simulink model "W09_E4_Bandwidth"  (R2024b)
settings: Solver=ode45  StartTime=0.0  StopTime=t_end  MaxStep=0.02  RelTol=1e-3
PreLoadFcn:
  | % W09_E4_Bandwidth 기본 파라미터 (모델을 열 때 자동 실행)
  | defs = { 'K',0.5 ; 'w_in',0.4 ; 't_end',120 ;
  |          'numG',1 ; 'denG',[1 2 1 0] };
  | for ii = 1:size(defs,1)
  |     if ~evalin('base', sprintf('exist(''%s'',''var'')', defs{ii,1}))
  |         assignin('base', defs{ii,1}, defs{ii,2});
  |     end
  | end
  | clear defs ii
values from neighbouring files (symbols this model uses):
  K = 0.5    [W09_02_pm_to_time.m]    (also in W09_03_run_simulink.m; W09_07_examples.m)
  w_in = w_list(i)    [W09_07_examples.m]
undefined symbols (not defined in the file or in its folder): denG, numG
settings Model: Creator=admin  LastModifiedBy=admin

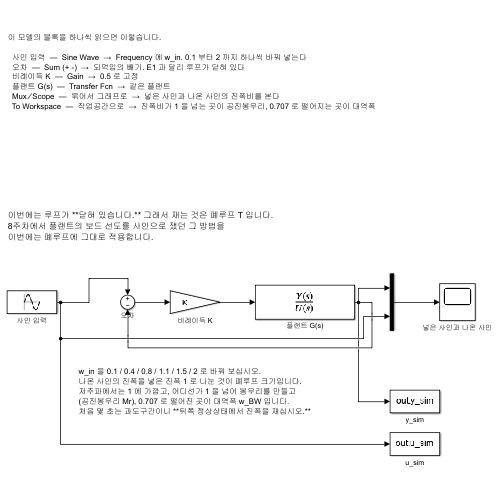
[thumbnail: Simulink's stored preview of the top-level diagram]
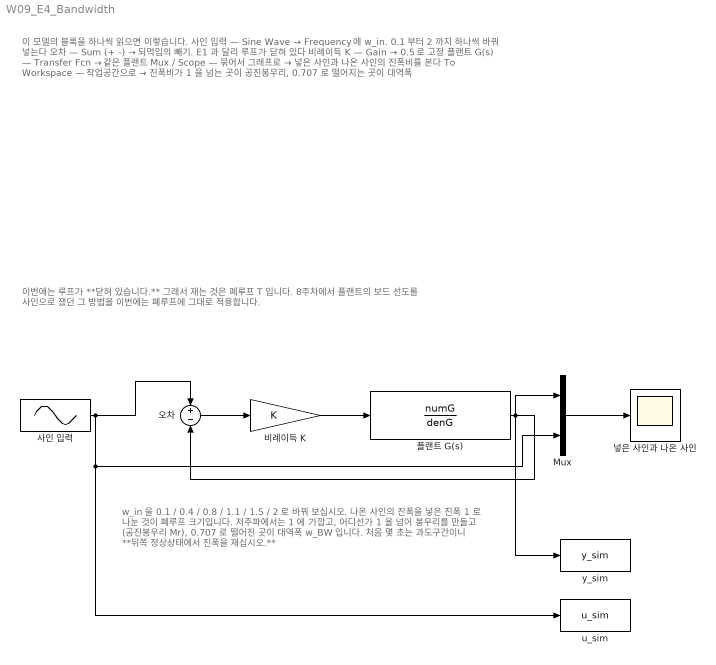
== system W09_E4_Bandwidth ==
  note: 이번에는 루프가 **닫혀 있습니다.** 그래서 재는 것은 폐루프 T 입니다.
      | 8주차에서 플랜트의 보드 선도를 사인으로 쟀던 그 방법을
      | 이번에는 폐루프에 그대로 적용합니다.
  note: w_in 을 0.1 / 0.4 / 0.8 / 1.1 / 1.5 / 2 로 바꿔 보십시오.
      | 나온 사인의 진폭을 넣은 진폭 1 로 나눈 것이 폐루프 크기입니다.
      | 저주파에서는 1 에 가깝고, 어디선가 1 을 넘어 봉우리를 만들고
      | (공진봉우리 Mr), 0.707 로 떨어진 곳이 대역폭 w_BW 입니다.
      | 처음 몇 초는 과도구간이니 **뒤쪽 정상상태에서 진폭을 재십시오.**
  note: 이 모델의 블록을 하나씩 읽으면 이렇습니다.
      |
      |   사인 입력  —  Sine Wave  →  Frequency 에 w_in. 0.1 부터 2 까지 하나씩 바꿔 넣는다
      |   오차  —  Sum (+ -)  →  되먹임의 빼기. E1 과 달리 루프가 닫혀 있다
      |   비례이득 K  —  Gain  →  0.5 로 고정
      |   플랜트 G(s)  —  Transfer Fcn  →  같은 플랜트
      |   Mux ∕ Scope  —  묶어서 그래프로  →  넣은 사인과 나온 사인의 진폭비를 본다
      |   To Workspace  —  작업공간으로  →  진폭비가 1 을 넘는 곳이 공진봉우리, 0.707 로 떨어지는 곳이 대역폭
  Mux : Mux  Inputs=2
  u_sim : ToWorkspace  VariableName=u_sim  SaveFormat=Timeseries  SampleTime=-1
  y_sim : ToWorkspace  VariableName=y_sim  SaveFormat=Timeseries  SampleTime=-1
  넣은 사인과 나온 사인 : Scope
  비례이득 K : Gain  Gain=K
  사인 입력 : Sin  Frequency=w_in  SampleTime=0
  오차 : Sum  Inputs=+-
  플랜트 G(s) : TransferFcn  Numerator=numG  Denominator=denG
  wires:
  사인 입력/1 -> Mux/2, u_sim/1, 오차/1
  오차/1 -> 비례이득 K/1
  비례이득 K/1 -> 플랜트 G(s)/1
  플랜트 G(s)/1 -> 오차/2, Mux/1, y_sim/1
  Mux/1 -> 넣은 사인과 나온 사인/1
